simulink model "v1_0_3_sim_fsfc"  (R2024a)
settings: Solver=FixedStepAuto  StartTime=0.0  StopTime=inf  FixedStep=Ts_pwm  RelTol=1e-3
values from neighbouring files (symbols this model uses):
  A = [ -Rs/L,           0,                  0 ... (first row only)    [mcb_pmsm_fsfb_f28379d_param.m]    (also in v0_pmsm_fsfb_sim_for_flipsky_.m = [; v1_0_3_sim_param_fsfc.m = [)
  B = [ 1/L,  0 ... (first row only)    [mcb_pmsm_fsfb_f28379d_param.m]    (also in v0_pmsm_fsfb_sim_for_flipsky_.m = [; v1_0_3_sim_param_fsfc.m = [)
  Bv = pmsm.B    [mcb_pmsm_foc_qep_f28379d_SIUnit_data.m]    (also in mcb_pmsm_fsfb_f28379d_param.m = 2.636e-06; v0_pmsm_fsfb_sim_for_flipsky_.m = 9.444e-05; v1_0_3_sim_param_fsfc.m = 9.444e-05)
  C = [ 1, 0, 0 ... (first row only)    [mcb_pmsm_fsfb_f28379d_param.m]    (also in v0_pmsm_fsfb_sim_for_flipsky_.m = [; v1_0_3_sim_param_fsfc.m = [)
  J = 7.061e-6    (= 7.061e-06)    [mcb_pmsm_fsfb_f28379d_param.m]    (also in v0_pmsm_fsfb_sim_for_flipsky_.m = 0.00036179; v1_0_3_sim_param_fsfc.m = 0.00036179)
  Ki = -Ka_fsfb(2)    [mcb_pmsm_foc_qep_f28379d_SIUnit_data.m]    (also in mcb_pmsm_fsfb_f28379d_param.m = -K(:, n+1:end); v0_pmsm_fsfb_sim_for_flipsky_.m = -K(:, n+1:end); v1_0_3_sim_param_fsfc.m = -K(:, n+1:end))
  Kx = K(:, 1:n)    [mcb_pmsm_fsfb_f28379d_param.m]    (also in v0_pmsm_fsfb_sim_for_flipsky_.m; v1_0_3_sim_param_fsfc.m)
  L = Ld    (= 0.0002)    [mcb_pmsm_fsfb_f28379d_param.m]    (also in v0_pmsm_fsfb_sim_for_flipsky_.m = 0.0004; v1_0_3_sim_param_fsfc.m = 0.0013)
  Lambda_m = 0.01273    [mcb_pmsm_fsfb_f28379d_param.m]    (also in v0_pmsm_fsfb_sim_for_flipsky_.m = 0.0426; v1_0_3_sim_param_fsfc.m = 0.08627)
  P = 8    [mcb_pmsm_fsfb_f28379d_param.m]    (also in v0_pmsm_fsfb_sim_for_flipsky_.m; v1_0_3_sim_param_fsfc.m)
  Pk0 = 5e-4*diag([1e-3, 1e-2, 0.2, 0.01])    [v0_pmsm_fsfb_sim_for_flipsky_.m]    (also in v1_0_3_sim_param_fsfc.m)
  Qd = 1e-4*diag([0.5, 0.5, 5, 0.5])    [v0_pmsm_fsfb_sim_for_flipsky_.m]    (also in v1_0_3_sim_param_fsfc.m)
  R = Rs    (= 0.72)    [v0_pmsm_fsfb_sim_for_flipsky_.m]    (also in v1_0_3_sim_param_fsfc.m = 0.52)
  Rc = 56.33    [v0_pmsm_fsfb_sim_for_flipsky_.m]    (also in v1_0_3_sim_param_fsfc.m = 450)
  Rs = 0.3819    [mcb_pmsm_fsfb_f28379d_param.m]    (also in v0_pmsm_fsfb_sim_for_flipsky_.m = 0.72; v1_0_3_sim_param_fsfc.m = 0.52)
  Tc = 0.001    [v0_pmsm_fsfb_sim_for_flipsky_.m]    (also in v1_0_3_sim_param_fsfc.m)
  Ts = T_pwm    (= 5e-05)    [mcb_pmsm_foc_qep_f28379d_SIUnit_data.m]    (also in v0_pmsm_fsfb_sim_for_flipsky_.m = 0.0001; v1_0_3_sim_param_fsfc.m = 0.0001)
  Ts_ov = 1e-6    (= 1e-06)    [v0_pmsm_fsfb_sim_for_flipsky_.m]    (also in v1_0_3_sim_param_fsfc.m)
  Ts_pwm = 1/20000    (= 5e-05)    [mcb_pmsm_fsfb_f28379d_param.m]    (also in v0_pmsm_fsfb_sim_for_flipsky_.m = 0.0001; v1_0_3_sim_param_fsfc.m = 0.0001)
  Vdc = 24    [mcb_pmsm_fsfb_f28379d_param.m]    (also in v0_pmsm_fsfb_sim_for_flipsky_.m = 48*sqrt(3); v1_0_3_sim_param_fsfc.m = 150*sqrt(3))
  X03 = [0; 0; 0]    [v0_pmsm_fsfb_sim_for_flipsky_.m]    (also in v1_0_3_sim_param_fsfc.m)
  X04 = 1e-2*[1; 1; 1; 0]    [v0_pmsm_fsfb_sim_for_flipsky_.m]    (also in v1_0_3_sim_param_fsfc.m)
undefined symbols (not defined in the file or in its folder): Down, Up
libraries: spsMosfetLib x6, simulink x4, spsDCVoltageSourceLib x1, spsGroundLib x1, spsPermanentMagnetSynchronousMachineLib x1, spsThreePhaseVIMeasurementLib x1, spspowerguiLib x1, eeGeneralControl x1, spsSVPWMGenerator2LevelLib x1
(part 1 of 2)
settings Model: Creator=rotanakchhean  LastModifiedBy=rotanakchhean

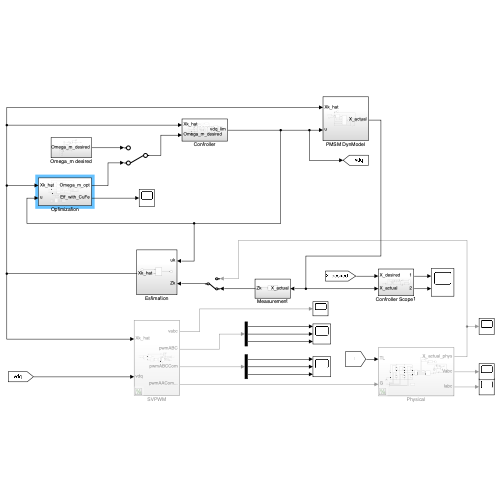
[thumbnail: Simulink's stored preview of the top-level diagram]
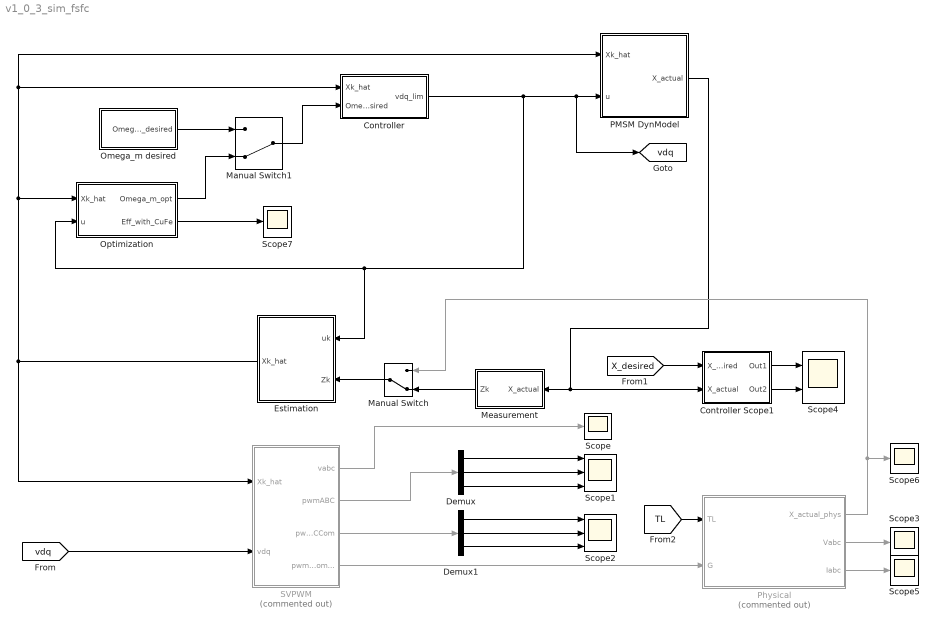
== system v1_0_3_sim_fsfc ==
  Controller : Subsystem
  Controller Scope1 : Subsystem
  Demux : Demux  Outputs=3
  Demux1 : Demux  Outputs=3
  Estimation : Subsystem
  Manual Switch : ManualSwitch  CurrentSetting=0
  Manual Switch1 : ManualSwitch  CurrentSetting=0
  Measurement : Subsystem
  Omega_m desired : Subsystem
  Optimization : Subsystem
  PMSM DynModel : Subsystem
  Physical : Subsystem  Commented=on
  SVPWM : Subsystem  Commented=on
  Scope{,3,5..7} (5 alike) : Scope
  Scope1 : Scope  NumInputPorts=3
  Scope2 : Scope  NumInputPorts=3
  Scope4 : Scope  NumInputPorts=2
  tag scope: vdq=global
  wires:
  Estimation/1(Xk_hat) -> Optimization/1(Xk_hat), PMSM DynModel/1(Xk_hat), Controller/1(Xk_hat), SVPWM/1(Xk_hat)
  SVPWM/1(vabc) -> Scope/1
  [vdq] -> SVPWM/2(vdq)
  Controller Scope1/2(Out2) -> Scope4/2
  Controller Scope1/1(Out1) -> Scope4/1
  [X_desired] -> Controller Scope1/1(X_desired)
  PMSM DynModel/1(X_actual) -> Measurement/1(X_actual), Controller Scope1/2(X_actual)
  SVPWM/2(pwmABC) -> Demux/1
  SVPWM/3(pwmABCCom) -> Demux1/1
  Demux/1 -> Scope1/1
  Demux/2 -> Scope1/2
  Demux/3 -> Scope1/3
  Demux1/1 -> Scope2/1
  Demux1/2 -> Scope2/2
  Demux1/3 -> Scope2/3
  SVPWM/4(pwmAACom...) -> Physical/2(G)
  [TL] -> Physical/1(TL)
  Physical/2(Vabc) -> Scope3/1
  Physical/3(Iabc) -> Scope5/1
  Physical/1(X_actual_phys) -> Manual Switch/1, Scope6/1
  Measurement/1(Zk) -> Manual Switch/2
  Manual Switch/1 -> Estimation/2(Zk)
  Optimization/2(Eff_with_CuFe) -> Scope7/1
  Controller/1(vdq_lim) -> Optimization/2(u), Estimation/1(uk), [vdq], PMSM DynModel/2(u)
  Omega_m desired/1(Omega_m_desired) -> Manual Switch1/1
  Optimization/1(Omega_m_opt) -> Manual Switch1/2
  Manual Switch1/1 -> Controller/2(Omega_m_desired)

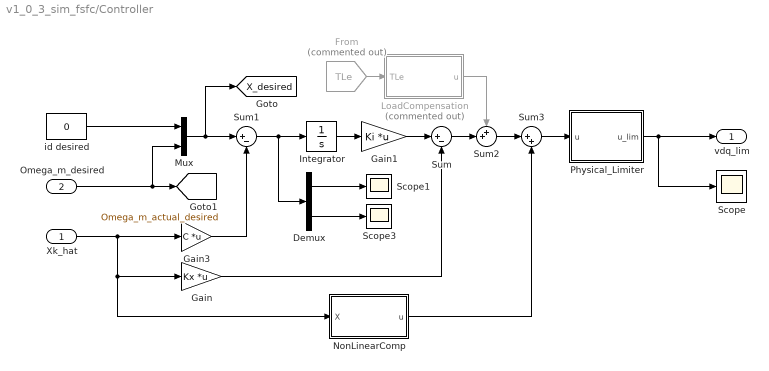
== system v1_0_3_sim_fsfc/Controller ==
  Xk_hat : Inport
  Omega_m_desired : Inport  Port=2
  Demux : Demux  Outputs=2
  From : From  Commented=on  GotoTag=TLe  TagVisibility=global
  Gain : Gain  Gain=Kx  Multiplication=Matrix(K*u)
  Gain1 : Gain  Gain=Ki  Multiplication=Matrix(K*u)
  Gain3 : Gain  Gain=C  Multiplication=Matrix(K*u)
  Integrator : Integrator
  LoadCompensation : MATLAB Function  Commented=on  TreatAsAtomicUnit=on
  Mux : Mux  Inputs=2
  NonLinearComp : MATLAB Function  TreatAsAtomicUnit=on
  Physical_Limiter : MATLAB Function  TreatAsAtomicUnit=on
  Scope : Scope
  Scope1 : Scope
  Scope3 : Scope
  Sum : Sum  Inputs=|+-
  Sum1 : Sum  Inputs=|+-
  Sum2 : Sum  Inputs=++|
  Sum3 : Sum  Inputs=|++
  id desired : Constant  Value=0
  vdq_lim : Outport
  tag scope: Omega_m_actual_desired=global, X_desired=global
  wires:
  Gain1/1 -> Sum/1
  NonLinearComp/1(u) -> Sum3/2
  Gain/1 -> Sum/2
  Sum1/1 -> Integrator/1, Demux/1
  Sum/1 -> Sum2/2
  Integrator/1 -> Gain1/1
  Gain3/1 -> Sum1/2
  Omega_m_desired/1 -> Mux/2, [Omega_m_actual_desired]
  id desired/1 -> Mux/1
  Physical_Limiter/1(u_lim) -> Scope/1, vdq_lim/1
  Sum3/1 -> Physical_Limiter/1(u)
  LoadCompensation/1(u) -> Sum2/1
  Xk_hat/1 -> Gain/1, NonLinearComp/1(X), Gain3/1
  Sum2/1 -> Sum3/1
  Demux/1 -> Scope1/1
  From/1 -> LoadCompensation/1(TLe)
  Demux/2 -> Scope3/1
  Mux/1 -> [X_desired], Sum1/1

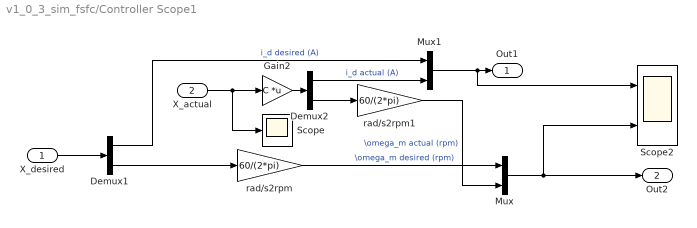
== system v1_0_3_sim_fsfc/Controller Scope1 ==
  X_desired : Inport
  X_actual : Inport  Port=2
  Demux1 : Demux  Outputs=2
  Demux2 : Demux  Outputs=2
  Gain2 : Gain  Gain=C  Multiplication=Matrix(K*u)
  Mux : Mux  Inputs=2
  Mux1 : Mux  Inputs=2
  Scope : Scope
  Scope2 : Scope  NumInputPorts=2
  rad/s2rpm : Gain  Gain=60/(2*pi)
  rad/s2rpm1 : Gain  Gain=60/(2*pi)
  Out1 : Outport
  Out2 : Outport  Port=2
  wires:
  X_actual/1 -> Scope/1, Gain2/1
  Demux1/1 -> Mux1/1  "i_d desired (A)"
  Demux2/1 -> Mux1/2  "i_d actual (A)"
  Gain2/1 -> Demux2/1
  Mux1/1 -> Scope2/1, Out1/1
  X_desired/1 -> Demux1/1
  Demux2/2 -> rad/s2rpm1/1
  Demux1/2 -> rad/s2rpm/1
  Mux/1 -> Scope2/2, Out2/1
  rad/s2rpm/1 -> Mux/1  "\\omega_m desired (rpm)"
  rad/s2rpm1/1 -> Mux/2  "\\omega_m actual (rpm)"

== system v1_0_3_sim_fsfc/Estimation ==
  uk : Inport
  Zk : Inport  Port=2
  EKF Estimation : Subsystem
  Xk_hat : Outport
  wires:
  EKF Estimation/1(Xk_hat) -> Xk_hat/1
  Zk/1 -> EKF Estimation/2(Zk)
  uk/1 -> EKF Estimation/1(uk)

== system v1_0_3_sim_fsfc/Measurement ==
  X_actual : Inport
  Measurement Noise : Subsystem
  Zk : Outport
  wires:
  X_actual/1 -> Measurement Noise/1(In2)
  Measurement Noise/1(Zk) -> Zk/1

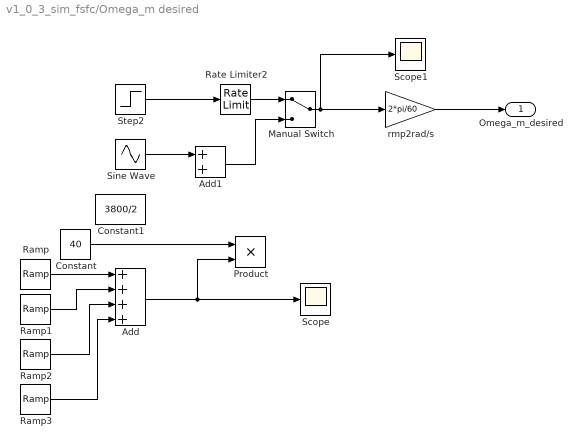
== system v1_0_3_sim_fsfc/Omega_m desired ==
  Add : Sum  Inputs=++++
  Add1 : Sum
  Constant : Constant  Value=40
  Constant1 : Constant  Value=3800/2
  Manual Switch : ManualSwitch
  Product : Product
  Ramp : simulink/Sources/Ramp  slope=1  start=5  InitialOutput=0
  Ramp1 : simulink/Sources/Ramp  slope=-1  start=15  InitialOutput=0
  Ramp2 : simulink/Sources/Ramp  slope=-1  start=35  InitialOutput=0
  Ramp3 : simulink/Sources/Ramp  slope=1  start=45  InitialOutput=0
  Rate Limiter2 : RateLimiter  RisingSlewLimit=700  FallingSlewLimit=-700  SampleTimeMode=inherited
  Scope : Scope
  Scope1 : Scope
  Sine Wave : Sin  Amplitude=3800  Frequency=2*pi*0.25  SampleTime=0
  Step2 : Step  Time=0  After=2200  SampleTime=0
  rmp2rad/s : Gain  Gain=2*pi/60
  Omega_m_desired : Outport
  wires:
  Rate Limiter2/1 -> Manual Switch/1
  rmp2rad/s/1 -> Omega_m_desired/1
  Sine Wave/1 -> Add1/1
  Step2/1 -> Rate Limiter2/1
  Ramp/1 -> Add/1
  Ramp1/1 -> Add/2
  Ramp2/1 -> Add/3
  Add/1 -> Product/2, Scope/1
  Ramp3/1 -> Add/4
  Constant/1 -> Product/1
  Manual Switch/1 -> Scope1/1, rmp2rad/s/1
  Add1/1 -> Manual Switch/2

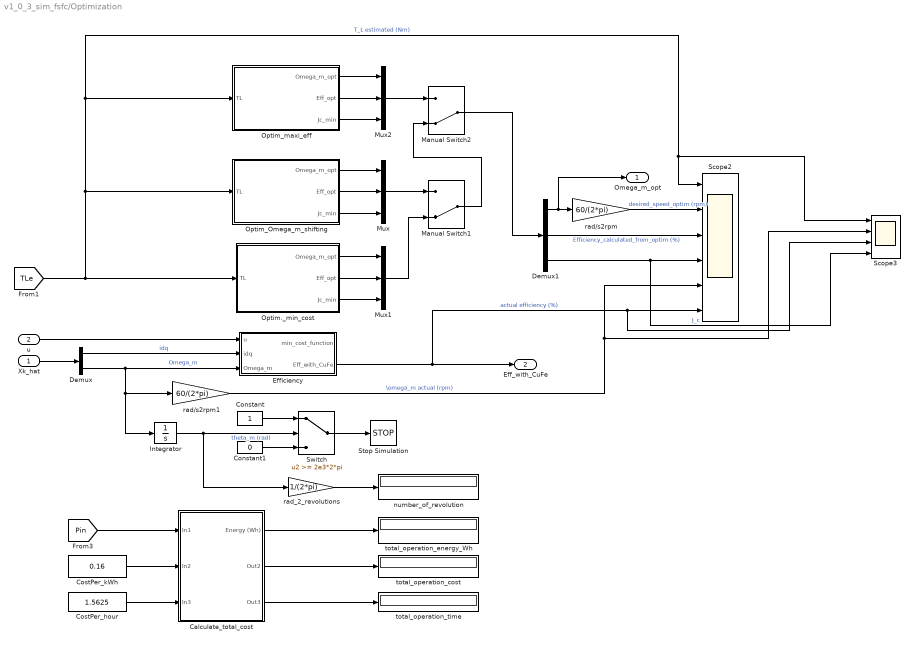
== system v1_0_3_sim_fsfc/Optimization ==
  Xk_hat : Inport
  u : Inport  Port=2
  Calculate_total_cost : Subsystem
  Constant : Constant
  Constant1 : Constant  Value=0
  CostPer_hour : Constant  Value=1.5625
  CostPer_kWh : Constant  Value=0.16
  Demux : Demux  Outputs=[2, 1]
  Demux1 : Demux  Outputs=3
  Efficiency : Subsystem
  Integrator : Integrator
  Manual Switch1 : ManualSwitch  CurrentSetting=0
  Manual Switch2 : ManualSwitch  CurrentSetting=0
  Mux : Mux  Inputs=3
  Mux1 : Mux  Inputs=3
  Mux2 : Mux  Inputs=3
  Optim._min_cost : MATLAB Function  TreatAsAtomicUnit=on
  Optim_Omega_m_shifting : MATLAB Function  TreatAsAtomicUnit=on
  Optim_maxi_eff : MATLAB Function  TreatAsAtomicUnit=on
  Scope2 : Scope  NumInputPorts=6
  Scope3 : Scope  NumInputPorts=4
  Stop Simulation : Stop
  Switch : Switch  Threshold=2e3*2*pi  SaturateOnIntegerOverflow=off  InputSameDT=off
  number_of_revolution : Display
  rad/s2rpm : Gain  Gain=60/(2*pi)
  rad/s2rpm1 : Gain  Gain=60/(2*pi)
  rad_2_revolutions : Gain  Gain=1/(2*pi)
  total_operation_cost : Display
  total_operation_energy_Wh : Display
  total_operation_time : Display
  Omega_m_opt : Outport
  Eff_with_CuFe : Outport  Port=2
  wires:
  Xk_hat/1 -> Demux/1
  u/1 -> Efficiency/1(u)
  Demux/1 -> Efficiency/2(idq)  "idq"
  Demux/2 -> Efficiency/3(Omega_m), Integrator/1, rad/s2rpm1/1  "Omega_m"
  rad/s2rpm/1 -> Scope2/2  "desired_speed_optim (rpm)"
  Efficiency/2(Eff_with_CuFe) -> Scope3/3, Scope2/6, Eff_with_CuFe/1  "actual efficiency (%)"
  Demux1/1 -> rad/s2rpm/1, Omega_m_opt/1
  [TLe] -> Optim._min_cost/1(TL), Optim_Omega_m_shifting/1(TL), Scope2/1, Scope3/1, Optim_maxi_eff/1(TL)  "T_L estimated (Nm)"
  rad/s2rpm1/1 -> Scope2/5, Scope3/2  "\\omega_m actual (rpm)"
  Integrator/1 -> Switch/2, rad_2_revolutions/1  "theta_m (rad)"
  Constant1/1 -> Switch/3
  Constant/1 -> Switch/1
  Calculate_total_cost/2(Out2) -> total_operation_cost/1
  [Pin] -> Calculate_total_cost/1(In1)
  CostPer_kWh/1 -> Calculate_total_cost/2(In2)
  CostPer_hour/1 -> Calculate_total_cost/3(In3)
  Calculate_total_cost/1(Energy (Wh)) -> total_operation_energy_Wh/1
  Calculate_total_cost/3(Out3) -> total_operation_time/1
  Optim_Omega_m_shifting/3(Jc_min) -> Mux/3
  Optim_Omega_m_shifting/2(Eff_opt) -> Mux/2
  Optim._min_cost/2(Eff_opt) -> Mux1/2
  Optim._min_cost/1(Omega_m_opt) -> Mux1/1
  Optim._min_cost/3(Jc_min) -> Mux1/3
  Mux/1 -> Manual Switch1/1
  Mux1/1 -> Manual Switch1/2
  Optim_Omega_m_shifting/1(Omega_m_opt) -> Mux/1
  Demux1/3 -> Scope3/4, Scope2/4  "J_c"
  rad_2_revolutions/1 -> number_of_revolution/1
  Optim_maxi_eff/1(Omega_m_opt) -> Mux2/1
  Optim_maxi_eff/2(Eff_opt) -> Mux2/2
  Optim_maxi_eff/3(Jc_min) -> Mux2/3
  Mux2/1 -> Manual Switch2/1
  Manual Switch1/1 -> Manual Switch2/2
  Manual Switch2/1 -> Demux1/1
  Demux1/2 -> Scope2/3  "Efficiency_calculated_from_optim (%)"
  Switch/1 -> Stop Simulation/1

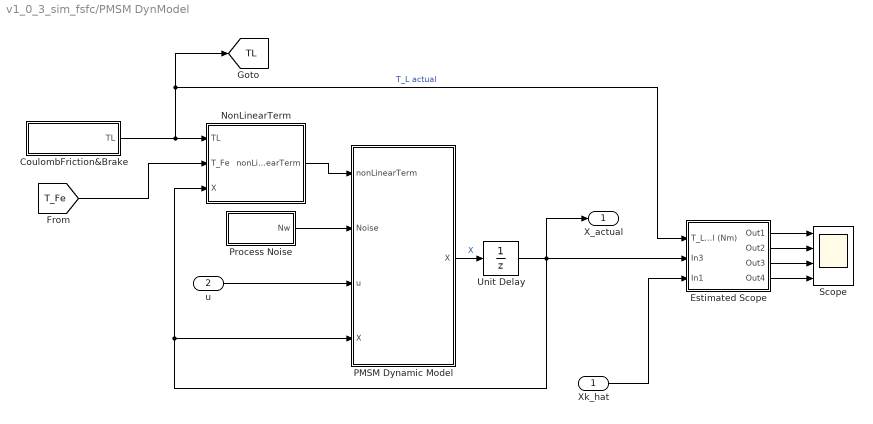
== system v1_0_3_sim_fsfc/PMSM DynModel ==
  Xk_hat : Inport
  u : Inport  Port=2
  CoulombFriction&Brake : Subsystem
  Estimated Scope : Subsystem
  NonLinearTerm : MATLAB Function  TreatAsAtomicUnit=on
  PMSM Dynamic Model : MATLAB Function  TreatAsAtomicUnit=on
  Process Noise : Subsystem
  Scope : Scope  NumInputPorts=4
  Unit Delay : UnitDelay  InitialCondition=X03  SampleTime=-1  HasFrameUpgradeWarning=on
  X_actual : Outport
  tag scope: TL=global
  wires:
  Xk_hat/1 -> Estimated Scope/3(In1)
  Estimated Scope/4(Out4) -> Scope/4
  Estimated Scope/2(Out2) -> Scope/2
  Estimated Scope/1(Out1) -> Scope/1
  Unit Delay/1 -> NonLinearTerm/3(X), PMSM Dynamic Model/4("X "), X_actual/1, Estimated Scope/2(In3)
  Process Noise/1(Nw) -> PMSM Dynamic Model/2(Noise)
  PMSM Dynamic Model/1(X) -> Unit Delay/1  "X"
  NonLinearTerm/1(nonLinearTerm) -> PMSM Dynamic Model/1(nonLinearTerm)
  Estimated Scope/3(Out3) -> Scope/3
  CoulombFriction&Brake/1(TL) -> [TL], Estimated Scope/1(T_L actual (Nm)), NonLinearTerm/1(TL)  "T_L actual"
  u/1 -> PMSM Dynamic Model/3(u)
  [T_Fe] -> NonLinearTerm/2(T_Fe)

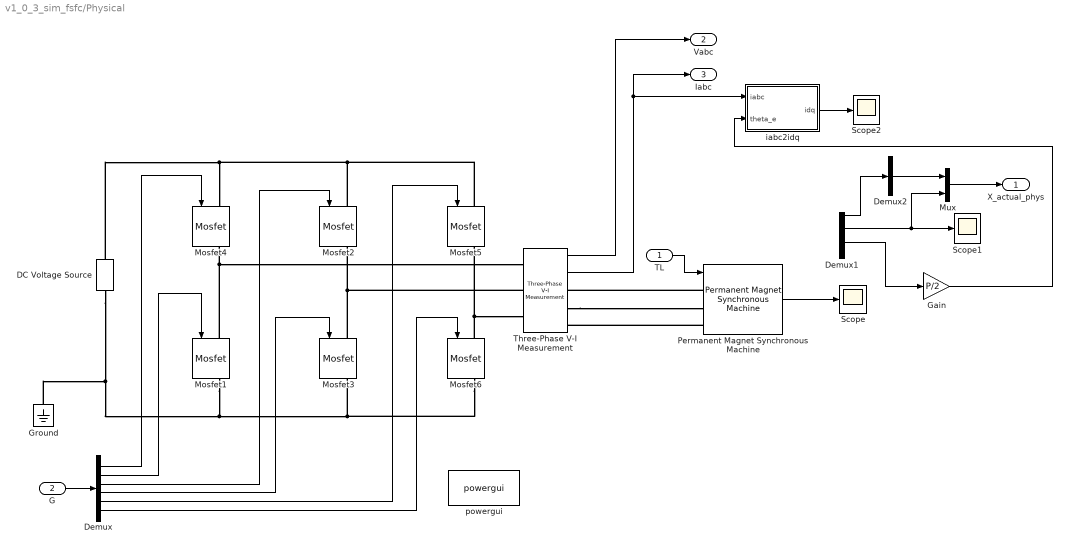
== system v1_0_3_sim_fsfc/Physical ==
  TL : Inport
  G : Inport  Port=2
  DC Voltage Source : spsDCVoltageSourceLib/DC Voltage Source  Amplitude=Vdc  Measurements=None
  Demux : Demux  Outputs=6
  Demux1 : Demux  Outputs=[10, 1, 1, 1]
  Demux2 : Demux  Outputs=[3, 2, 5]
  Gain : Gain  Gain=P/2
  Ground : spsGroundLib/Ground  LConnTagsString=a
  Mosfet{1..6} (6 alike) : spsMosfetLib/Mosfet  Ron=0.001  Lon=0  Rd=0.001  Vfd=0.6  IC=0  Rs=1e5  Cs=inf  Measurements=on
  Mux : Mux  Inputs=2
  Permanent Magnet Synchronous Machine : spsPermanentMagnetSynchronousMachineLib/Permanent Magnet Synchronous Machine  NbPhases=3  FluxDistribution=Sinusoidal  RotorType=Round  MechanicalLoad=Torque Tm  PresetModel=No  ShowDetailedParameters=on  MeasurementBus=off  Resistance=R  Inductance=8.5e-3  dqInductances=[8.5e-3,8.5e-3]  La=L  MachineConstant=Flux linkage established by magnets (V.s)  Flux=Lambda_m  VoltageCst=62.5906  TorqueCst=0.51762  Flat=120  Mechanical=[J Bv P/2 1e-3]  PolePairs=4  InitialConditions=[0,0, 0,0]  InitialConditions5ph=[0 0 0 0 0 0]  RefAngle=90 degrees behind phase A axis (modified Park)  IterativeDiscreteModel=Trapezoidal non iterative  TsBlock=-1  TsPowergui=0
  Scope : Scope
  Scope1 : Scope
  Scope2 : Scope
  Three-Phase V-I Measurement : spsThreePhaseVIMeasurementLib/Three-Phase V-I Measurement  VoltageMeasurement=phase-to-phase  SetLabelV=off  LabelV=Vabc  Vpu=off  VpuLL=off  CurrentMeasurement=yes  SetLabelI=off  LabelI=Iabc  Ipu=off  Pbase=100e6  Vbase=500e3  OutputType=Complex  PhasorSimulation=off  PSBequivalent=0
  iabc2idq : Subsystem
  powergui : spspowerguiLib/powergui  Priority=1  SimulationMode=Continuous  SampleTime=50e-6  frequency=60  Iterations=50  frequencyindice=0  Pbase=100e6  ErrMax=1e-4  UnitsV=kV  UnitsW=MW  buscounter=0  FunctionMessages=off  echomessages=off  EnableUseOfTLC=off  CurrentSourceSwitches=off  DisableSnubberDevices=off  DisableRonSwitches=off  DisableVfSwitches=off  DisplayEquations=off  AutomaticDiscreteSolvers=off  SolverType=Tustin/Backward Euler (TBE)  Interpol=off  ExternalGateDelay=off  methode=off  Ts=100  x0status=blocks  SPID=on  SwTol=0  HookPort=off  NonlinearTolerance=1e-4  nMaxIteration=100  ContinueOnMaxIteration=off  RestoreLinks=warning  ResistiveCurrentMeasurement=off  Frange=[0:2:500]  Ylog=off  Xlog=on  ShowGrid=off  save=off  variable=ZData  structure=0  ZoomFFT=off  StartTime=0.0  cycles=1  DisplayStyle=1  fundamental=60  FreqAxis=off  MaxFrequency=1000  frequencyindicesteady=1  RmsSteady=1  display=off
  X_actual_phys : Outport
  Vabc : Outport  Port=2
  Iabc : Outport  Port=3
  wires:
  G/1 -> Demux/1
  Demux/1 -> Mosfet4/1
  Demux/2 -> Mosfet1/1
  Demux/3 -> Mosfet2/1
  Demux/4 -> Mosfet3/1
  Demux/5 -> Mosfet5/1
  Demux/6 -> Mosfet6/1
  TL/1 -> Permanent Magnet Synchronous Machine/1
  Three-Phase V-I Measurement/2 -> Iabc/1, iabc2idq/1(iabc)
  Three-Phase V-I Measurement/1 -> Vabc/1
  Permanent Magnet Synchronous Machine/1 -> Scope/1
  Demux1/2 -> Scope1/1, Mux/2
  Demux1/3 -> Gain/1
  Gain/1 -> iabc2idq/2(theta_e)
  iabc2idq/1(idq) -> Scope2/1
  Demux1/1 -> Demux2/1
  Demux2/2 -> Mux/1
  Mux/1 -> X_actual_phys/1
  connections:
  DC Voltage Source/RConn1 -- Mosfet5/LConn1 -- Mosfet2/LConn1 -- Mosfet4/LConn1
  Mosfet1/RConn1 -- Ground/LConn1 -- DC Voltage Source/LConn1 -- Mosfet3/RConn1 -- Mosfet6/RConn1
  Mosfet3/LConn1 -- Three-Phase V-I Measurement/LConn2 -- Mosfet2/RConn1
  Mosfet6/LConn1 -- Mosfet5/RConn1 -- Three-Phase V-I Measurement/LConn3
  Mosfet1/LConn1 -- Mosfet4/RConn1 -- Three-Phase V-I Measurement/LConn1
  Permanent Magnet Synchronous Machine/LConn1 -- Three-Phase V-I Measurement/RConn1
  Three-Phase V-I Measurement/RConn2 -- Permanent Magnet Synchronous Machine/LConn2
  Permanent Magnet Synchronous Machine/LConn3 -- Three-Phase V-I Measurement/RConn3

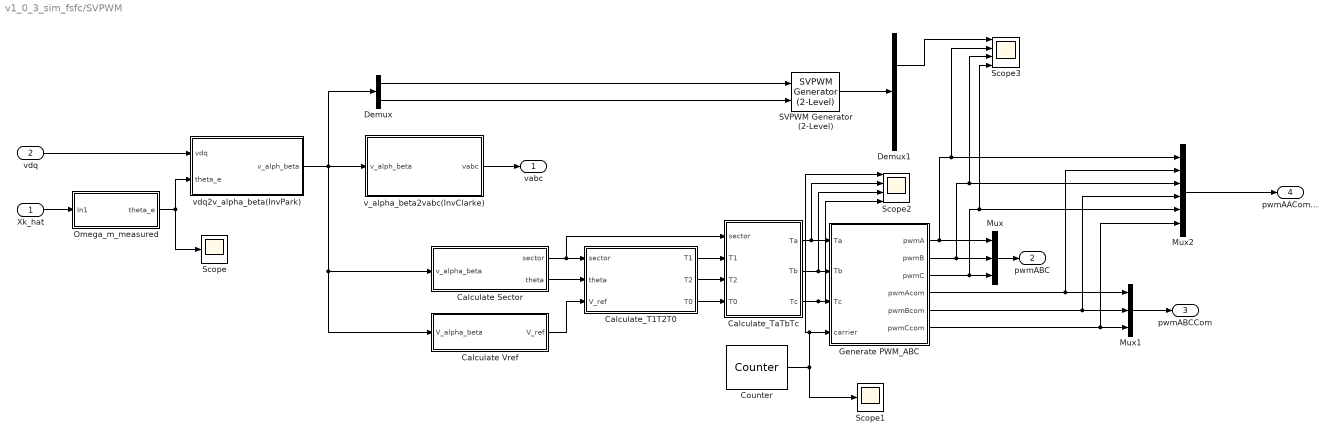
== system v1_0_3_sim_fsfc/SVPWM ==
  Xk_hat : Inport
  vdq : Inport  Port=2
  Calculate Sector : MATLAB Function  TreatAsAtomicUnit=on
  "Calculate Vref " : MATLAB Function  TreatAsAtomicUnit=on
  Calculate_T1T2T0 : MATLAB Function  TreatAsAtomicUnit=on
  Calculate_TaTbTc : MATLAB Function  TreatAsAtomicUnit=on
  Counter : eeGeneralControl/Counter  CarrCount=Up-Down  Range=[0 1]  Tper=Ts_pwm/2  Tdelay=0  Ts=Ts_ov
      settings: LibrarySourceBlock=ee_sl_lib/General Control/Counter
  Demux : Demux  Outputs=2
  Demux1 : Demux  Outputs=6
  Generate PWM_ABC : MATLAB Function  TreatAsAtomicUnit=on
  Mux : Mux  Inputs=3
  Mux1 : Mux  Inputs=3
  Mux2 : Mux  Inputs=6
  Omega_m_measured : Subsystem
  SVPWM Generator (2-Level) : spsSVPWMGenerator2LevelLib/SVPWM Generator (2-Level)  InputType=alpha-beta components  SwitchingPattern=Pattern #1  Fc=1e4  ParUref=[0.8 -30 50]  Ts=0
  Scope : Scope
  Scope1 : Scope
  Scope2 : Scope  NumInputPorts=4
  Scope3 : Scope  NumInputPorts=4
  v_alpha_beta2vabc(InvClarke) : MATLAB Function  TreatAsAtomicUnit=on
  vdq2v_alpha_beta(InvPark) : MATLAB Function  TreatAsAtomicUnit=on
  vabc : Outport
  pwmABC : Outport  Port=2
  pwmABCCom : Outport  Port=3
  pwmAACom... : Outport  Port=4
  wires:
  vdq/1 -> vdq2v_alpha_beta(InvPark)/1(vdq)
  Omega_m_measured/1(theta_e) -> Scope/1, vdq2v_alpha_beta(InvPark)/2(theta_e)
  v_alpha_beta2vabc(InvClarke)/1(vabc) -> vabc/1
  Xk_hat/1 -> Omega_m_measured/1(In1)
  Calculate_T1T2T0/1(T1) -> Calculate_TaTbTc/2(T1)
  "Calculate Vref "/1(V_ref) -> Calculate_T1T2T0/3(V_ref)
  Calculate_T1T2T0/2(T2) -> Calculate_TaTbTc/3(T2)
  Calculate_T1T2T0/3(T0) -> Calculate_TaTbTc/4(T0)
  Calculate_TaTbTc/1(Ta) -> Scope2/2, Generate PWM_ABC/1(Ta)
  Calculate_TaTbTc/2(Tb) -> Scope2/3, Generate PWM_ABC/2(Tb)
  Calculate_TaTbTc/3(Tc) -> Scope2/4, Generate PWM_ABC/3(Tc)
  Counter/1 -> Scope1/1, Generate PWM_ABC/4(carrier), Scope2/1
  Calculate Sector/2(theta) -> Calculate_T1T2T0/2(theta)
  Calculate Sector/1(sector) -> Calculate_T1T2T0/1(sector), Calculate_TaTbTc/1(sector)
  Generate PWM_ABC/1(pwmA) -> Mux/1, Mux2/1, Scope3/2
  Generate PWM_ABC/2(pwmB) -> Mux/2, Mux2/3, Scope3/3
  Generate PWM_ABC/3(pwmC) -> Mux/3, Scope3/4, Mux2/5
  Generate PWM_ABC/5(pwmBcom) -> Mux1/2, Mux2/4
  Generate PWM_ABC/6(pwmCcom) -> Mux1/3, Mux2/6
  Generate PWM_ABC/4(pwmAcom) -> Mux1/1, Mux2/2
  Mux1/1 -> pwmABCCom/1
  Mux/1 -> pwmABC/1
  Demux/1 -> SVPWM Generator (2-Level)/1
  Demux/2 -> SVPWM Generator (2-Level)/2
  vdq2v_alpha_beta(InvPark)/1(v_alph_beta) -> "Calculate Vref "/1(V_alpha_beta), Calculate Sector/1(v_alpha_beta), v_alpha_beta2vabc(InvClarke)/1(v_alph_beta), Demux/1
  SVPWM Generator (2-Level)/1 -> Demux1/1
  Demux1/2 -> Scope3/1
  Mux2/1 -> pwmAACom.../1

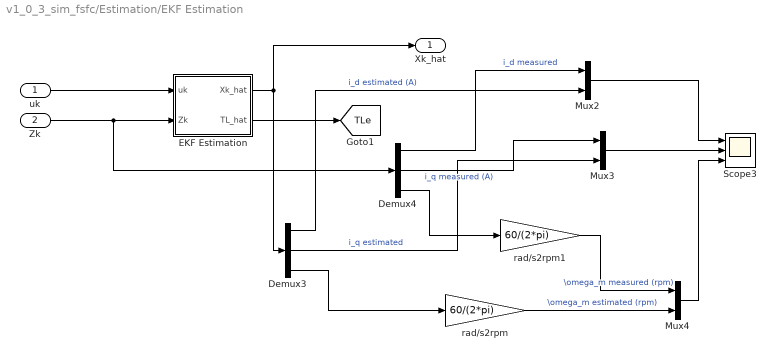
== system v1_0_3_sim_fsfc/Estimation/EKF Estimation ==
  uk : Inport
  Zk : Inport  Port=2
  Demux3 : Demux  Outputs=3
  Demux4 : Demux  Outputs=3
  EKF Estimation : Subsystem
  Mux2 : Mux  Inputs=2
  Mux3 : Mux  Inputs=2
  Mux4 : Mux  Inputs=2
  Scope3 : Scope  NumInputPorts=3
  rad/s2rpm : Gain  Gain=60/(2*pi)
  rad/s2rpm1 : Gain  Gain=60/(2*pi)
  Xk_hat : Outport
  tag scope: TLe=global
  wires:
  uk/1 -> EKF Estimation/1(uk)
  Demux3/3 -> rad/s2rpm/1
  EKF Estimation/1(Xk_hat) -> Xk_hat/1, Demux3/1
  Demux4/2 -> Mux3/1  "i_q measured (A)"
  Mux3/1 -> Scope3/2
  Demux3/1 -> Mux2/2  "i_d estimated (A)"
  Zk/1 -> Demux4/1, EKF Estimation/2(Zk)
  Demux4/3 -> rad/s2rpm1/1
  Mux2/1 -> Scope3/1
  Demux3/2 -> Mux3/2  "i_q estimated"
  EKF Estimation/2(TL_hat) -> [TLe]
  Demux4/1 -> Mux2/1  "i_d measured"
  Mux4/1 -> Scope3/3
  rad/s2rpm/1 -> Mux4/2  "\\omega_m estimated (rpm)"
  rad/s2rpm1/1 -> Mux4/1  "\\omega_m measured (rpm)"

== system v1_0_3_sim_fsfc/Measurement/Measurement Noise ==
  In2 : Inport
  Constant1 : Constant  Value=0.5
  Constant2 : Constant  Value=0.5
  Constant3 : Constant  Value=2
  "Measurement Noise " : MATLAB Function  TreatAsAtomicUnit=on
  Sum4 : Sum  Inputs=|++
  Zk : Outport
  wires:
  "Measurement Noise "/1(Nv) -> Sum4/2
  Constant2/1 -> "Measurement Noise "/2(Viq)
  Constant1/1 -> "Measurement Noise "/1(Vid)
  Constant3/1 -> "Measurement Noise "/3(Vwm)
  Sum4/1 -> Zk/1
  In2/1 -> Sum4/1

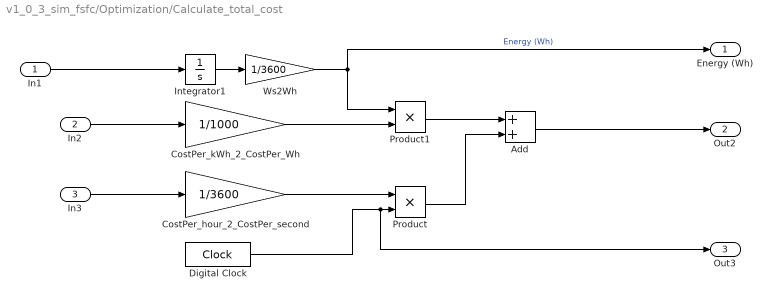
== system v1_0_3_sim_fsfc/Optimization/Calculate_total_cost ==
  In1 : Inport
  In2 : Inport  Port=2
  In3 : Inport  Port=3
  Add : Sum
  CostPer_hour_2_CostPer_second : Gain  Gain=1/3600
  CostPer_kWh_2_CostPer_Wh : Gain  Gain=1/1000
  Digital Clock : DigitalClock
  Integrator1 : Integrator
  Product : Product
  Product1 : Product
  Ws2Wh : Gain  Gain=1/3600
  Energy (Wh) : Outport
  Out2 : Outport  Port=2
  Out3 : Outport  Port=3
  wires:
  In1/1 -> Integrator1/1
  Add/1 -> Out2/1
  In3/1 -> CostPer_hour_2_CostPer_second/1
  CostPer_kWh_2_CostPer_Wh/1 -> Product1/2
  In2/1 -> CostPer_kWh_2_CostPer_Wh/1
  CostPer_hour_2_CostPer_second/1 -> Product/1
  Integrator1/1 -> Ws2Wh/1
  Product/1 -> Add/2
  Product1/1 -> Add/1
  Ws2Wh/1 -> Energy (Wh)/1, Product1/1  "Energy (Wh)"
  Digital Clock/1 -> Out3/1, Product/2

== system v1_0_3_sim_fsfc/Optimization/Efficiency ==
  u : Inport
  idq : Inport  Port=2
  Omega_m : Inport  Port=3
  Divide : Product  Inputs=*/
  MATLAB Function : MATLAB Function  TreatAsAtomicUnit=on
  Pin : Subsystem
  Pout : Subsystem
  Pout_hassan : Subsystem  Commented=on
  Scope : Scope
  min_cost_function : Outport
  Eff_with_CuFe : Outport  Port=2
  tag scope: Pin=global
  wires:
  idq/1 -> Pout/2(idq), Pin/1(idq)
  u/1 -> Pin/2(u)
  Pin/1(Pin) -> [Pin], Divide/2, Pout/3(Pin)
  Pout/1(Pout) -> Divide/1
  Divide/1 -> MATLAB Function/1("Eff ")
  Omega_m/1 -> Pout/1(Omega_m)
  MATLAB Function/1(Eff) -> Scope/1, Eff_with_CuFe/1

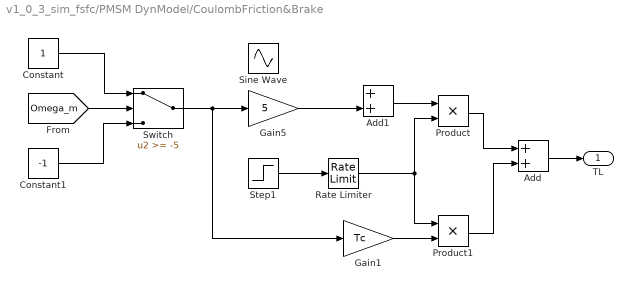
== system v1_0_3_sim_fsfc/PMSM DynModel/CoulombFriction&Brake ==
  Add : Sum
  Add1 : Sum
  Constant : Constant
  Constant1 : Constant  Value=-1
  Gain1 : Gain  Gain=Tc
  Gain5 : Gain  Gain=5
  Product : Product
  Product1 : Product
  Rate Limiter : RateLimiter  RisingSlewLimit=0.2  FallingSlewLimit=-0.2  SampleTimeMode=inherited
  Sine Wave : Sin  Amplitude=2  Frequency=2*pi*0.1  SampleTime=0
  Step1 : Step  Before=1  SampleTime=0
  Switch : Switch  Threshold=-5  SaturateOnIntegerOverflow=off  InputSameDT=off
  TL : Outport
  wires:
  Product/1 -> Add/1
  Switch/1 -> Gain5/1, Gain1/1
  Step1/1 -> Rate Limiter/1
  Gain1/1 -> Product1/2
  Product1/1 -> Add/2
  Add/1 -> TL/1
  Add1/1 -> Product/1
  Constant/1 -> Switch/1
  Constant1/1 -> Switch/3
  [Omega_m] -> Switch/2
  Rate Limiter/1 -> Product/2, Product1/1
  Gain5/1 -> Add1/2

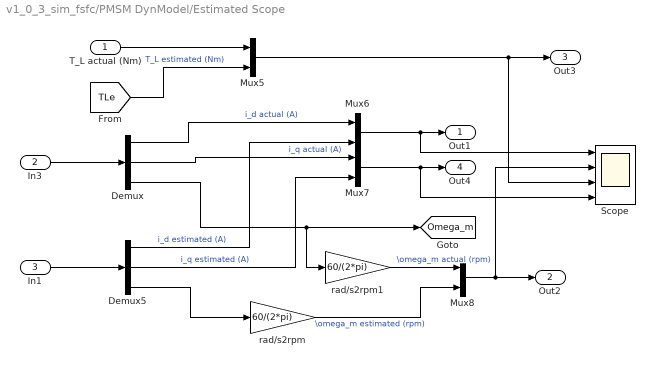
== system v1_0_3_sim_fsfc/PMSM DynModel/Estimated Scope ==
  T_L actual (Nm) : Inport
  In3 : Inport  Port=2
  In1 : Inport  Port=3
  Demux : Demux  Outputs=3
  Demux5 : Demux  Outputs=3
  Mux{5..8} (4 alike) : Mux  Inputs=2
  Scope : Scope  NumInputPorts=4
  rad/s2rpm : Gain  Gain=60/(2*pi)
  rad/s2rpm1 : Gain  Gain=60/(2*pi)
  Out1 : Outport
  Out2 : Outport  Port=2
  Out3 : Outport  Port=3
  Out4 : Outport  Port=4
  tag scope: Omega_m=global
  wires:
  In1/1 -> Demux5/1
  Demux5/3 -> rad/s2rpm/1
  [TLe] -> Mux5/2  "T_L estimated (Nm)"
  Mux6/1 -> Scope/1, Out1/1
  Mux5/1 -> Scope/3, Out3/1
  In3/1 -> Demux/1
  Demux/3 -> [Omega_m], rad/s2rpm1/1
  T_L actual (Nm)/1 -> Mux5/1
  Demux5/2 -> Mux7/2  "i_q estimated (A)"
  Demux5/1 -> Mux6/2  "i_d estimated (A)"
  Mux7/1 -> Scope/4, Out4/1
  Mux8/1 -> Scope/2, Out2/1
  Demux/1 -> Mux6/1  "i_d actual (A)"
  Demux/2 -> Mux7/1  "i_q actual (A)"
  rad/s2rpm/1 -> Mux8/2  "\\omega_m estimated (rpm)"
  rad/s2rpm1/1 -> Mux8/1  "\\omega_m actual (rpm)"

== system v1_0_3_sim_fsfc/PMSM DynModel/Process Noise ==
  Constant4 : Constant  Value=0.2e-4
  Constant5 : Constant  Value=0.2e-4
  Constant6 : Constant  Value=2e-4
  Process Noise : MATLAB Function  TreatAsAtomicUnit=on
  Nw : Outport
  wires:
  Constant5/1 -> Process Noise/2(Viq)
  Process Noise/1(Nw) -> Nw/1
  Constant4/1 -> Process Noise/1(Vid)
  Constant6/1 -> Process Noise/3(Vwm)

== system v1_0_3_sim_fsfc/Physical/iabc2idq ==
  iabc : Inport
  theta_e : Inport  Port=2
  i_alpha_beta2idq(FPark) : MATLAB Function  TreatAsAtomicUnit=on
  iabc2i_alpha_beta(FClarke) : MATLAB Function  TreatAsAtomicUnit=on
  idq : Outport
  wires:
  iabc/1 -> iabc2i_alpha_beta(FClarke)/1(iabc)
  iabc2i_alpha_beta(FClarke)/1(i_alpha_beta) -> i_alpha_beta2idq(FPark)/1(i_alpha_beta)
  i_alpha_beta2idq(FPark)/1(idq) -> idq/1
  theta_e/1 -> i_alpha_beta2idq(FPark)/2(theta_e)

== system v1_0_3_sim_fsfc/SVPWM/Omega_m_measured ==
  In1 : Inport
  Integrator : Integrator
  idqwm2wm : Gain  Gain=[0 0 1]  Multiplication=Matrix(K*u)
  wm2we : Gain  Gain=P/2
  theta_e : Outport
  wires:
  In1/1 -> idqwm2wm/1
  idqwm2wm/1 -> wm2we/1
  wm2we/1 -> Integrator/1
  Integrator/1 -> theta_e/1

== system v1_0_3_sim_fsfc/Estimation/EKF Estimation/EKF Estimation ==
  uk : Inport
  Zk : Inport  Port=2
  Demux : Demux
  MeasurementUpdateCorrect : MATLAB Function  TreatAsAtomicUnit=on
  Mux : Mux  Inputs=3
  TimeUpdatePredict : MATLAB Function  TreatAsAtomicUnit=on
  Unit Delay : UnitDelay  InitialCondition=Pk0  SampleTime=-1  HasFrameUpgradeWarning=on
  Unit Delay1 : UnitDelay  InitialCondition=X04  SampleTime=-1  HasFrameUpgradeWarning=on
  Unit Delay2 : UnitDelay  SampleTime=-1  HasFrameUpgradeWarning=on
  Xk_hat : Outport
  TL_hat : Outport  Port=2
  wires:
  uk/1 -> Unit Delay2/1
  TimeUpdatePredict/1(Pk1_p) -> MeasurementUpdateCorrect/2(Pk1_p)
  TimeUpdatePredict/2(Xk1_p) -> MeasurementUpdateCorrect/3(Xk1_p)
  Zk/1 -> MeasurementUpdateCorrect/1(Zk)
  MeasurementUpdateCorrect/2(Pk) -> Unit Delay/1
  Unit Delay/1 -> TimeUpdatePredict/3(Pk)
  MeasurementUpdateCorrect/1(Xk) -> Unit Delay1/1
  Unit Delay1/1 -> Demux/1, TimeUpdatePredict/2(Xk)
  Demux/3 -> Mux/3
  Demux/2 -> Mux/2
  Demux/1 -> Mux/1
  Mux/1 -> Xk_hat/1
  Demux/4 -> TL_hat/1
  Unit Delay2/1 -> TimeUpdatePredict/1(uk)

== system v1_0_3_sim_fsfc/Optimization/Efficiency/Pin ==
  idq : Inport
  u : Inport  Port=2
  Add : Sum
  Demux : Demux  Outputs=2
  Demux1 : Demux  Outputs=2
  Gain : Gain  Gain=1.5
  Product : Product
  Product1 : Product
  Pin : Outport
  wires:
  Product/1 -> Add/1
  Product1/1 -> Add/2
  Add/1 -> Gain/1
  Gain/1 -> Pin/1
  Demux1/1 -> Product/1  "id"
  Demux1/2 -> Product1/1  "iq"
  Demux/1 -> Product/2  "vd"
  Demux/2 -> Product1/2  "vq"
  u/1 -> Demux/1
  idq/1 -> Demux1/1

== system v1_0_3_sim_fsfc/Optimization/Efficiency/Pout ==
  Omega_m : Inport
  idq : Inport  Port=2
  Pin : Inport  Port=3
  Add : Sum  Inputs=----+
  P_Cu : MATLAB Function  TreatAsAtomicUnit=on
  P_Fe : MATLAB Function  TreatAsAtomicUnit=on
  Pm : MATLAB Function  TreatAsAtomicUnit=on
  Ps : Gain  Gain=0.01
  Pout : Outport
  tag scope: T_Fe=global
  wires:
  idq/1 -> Pm/1(idq), P_Fe/1(idq), P_Cu/1(idq)
  Pin/1 -> Ps/1, Add/5
  Ps/1 -> Add/4
  Pm/1(Pm) -> Add/3
  P_Fe/1(P_Fe) -> Add/2
  P_Cu/1(P_Cu) -> Add/1
  Add/1 -> Pout/1
  Omega_m/1 -> Pm/2(Omega_m), P_Cu/2(Omega_m), P_Fe/2(Omega_m)
  P_Fe/2(T_Fe) -> [T_Fe]

== system v1_0_3_sim_fsfc/Optimization/Efficiency/Pout_hassan ==
  Xk_hat : Inport
  Pin : Inport  Port=2
  Add : Sum  Inputs=+--
  Add1 : Sum  Inputs=--+--
  P_Cu : MATLAB Function  TreatAsAtomicUnit=on
  P_Fe : MATLAB Function  TreatAsAtomicUnit=on
  Pe : MATLAB Function  TreatAsAtomicUnit=on
  Pm : MATLAB Function  TreatAsAtomicUnit=on
  Ps : Gain  Gain=0.01
  Pout_with_Pe : Outport
  Pout_with_CuFe : Outport  Port=2
  wires:
  Pin/1 -> Add1/3, Ps/1
  Pe/1(Pe) -> Add/1
  Pm/1(Pm) -> Add/2, Add1/2
  Ps/1 -> Add1/1, Add/3
  Add/1 -> Pout_with_Pe/1
  Xk_hat/1 -> Pe/1(Xk_hat), Pm/1(Xk_hat), P_Fe/1(Xk_hat), P_Cu/1(Xk_hat)
  P_Cu/1(P_Cu) -> Add1/4
  P_Fe/1(P_Fe) -> Add1/5
  Add1/1 -> Pout_with_CuFe/1

== matlab function v1_0_3_sim_fsfc/Optimization/Optim_maxi_eff ==
  data: Omega_m_opt output; Eff_opt output; Jc_min output; TL input; Rc parameter; Lambda_m parameter; L parameter; P parameter; Rs parameter; Tc parameter; Bv parameter; J parameter
function [Omega_m_opt, Eff_opt, Jc_min] = fcn(TL, Rc, Lambda_m, L, P, Rs, Tc, Bv, J)

Omega_m_min = 500; %rpm
Omega_m_max = 4000; %rmp

Omega_m_min = Omega_m_min*2*pi/60; %rad/s
Omega_m_max = Omega_m_max*2*pi/60; %rad/s

Omega_e_min = (P/2)*Omega_m_min*2*pi/60; %rad/s
Omega_e_max = (P/2)*Omega_m_max*2*pi/60; %rad/s

%% Method 1

% Eff_opt = 0;
% Omega_e_opt = Omega_m_max*P/2;
% for Omega_m = linspace(Omega_m_min, Omega_m_max, 1000)
%     Omega_e = Omega_m*P/2;
%      Eff_opt_calc = Calculate_Eff(Omega_e, idq, u, Rc, Lambda_m, L, P, Rs, Tc, Bv);
%      if Eff_opt_calc > Eff_opt
%          Eff_opt = Eff_opt_calc;
%          Omega_e_opt = Omega_e;
%      end
% end
%% Method 2
% Omega_m_a = Omega_m_min;
% Omega_e_a = Omega_m_a*P/2;
% 
% Omega_m_b = Omega_m_max;
% Omega_e_b = Omega_m_b*P/2;
% 
% a = Omega_e_a;
% b = Omega_e_b;
% tol = 1e-4;
% 
% for i = 1:500
%     c = (a+b)/2;
%     dEff_c = Calculate_dEff(c, idq, u, Rc, Lambda_m, L, P, Rs, Tc, Bv);
% 
%     if abs(b - a) < tol
%         break;
%     end
% 
%     if dEff_c > 0
%         a = c;
%     else
%         b = c;
%     end
% 
% end
% Compute optimal Omega_m_opt
% Omega_e_opt = (a + b) / 2;
%% Method 3
alpha = 1;
theta_e = 2*pi*100;
Eff_1min = 10;
Eff_1max = 100;

Omega_e = linspace(0, 0, 1000);
Eff = linspace(0, 0, 1000);
i = 0;
for Omega_m = linspace(Omega_m_min, Omega_m_max, 1000)
    i = i+1;
    Omega_e(i) = Omega_m*P/2;
    Eff(i) = Calculate_Eff(Omega_e(i), TL, Rc, Lambda_m, L, P, Rs, Tc, Bv, J);
end
[Eff_max, Eff_idx] = max(Eff);
Omega_e_opt = Omega_e(Eff_idx);
Omega_m_opt = Omega_e_opt * 2 / P;
Eff_opt = Eff_max;
Jc_min = 0;

if Eff_opt < 0.2
    Eff_opt = 0.2;
elseif Eff_opt > 1
    Eff_opt = 1;
end
Eff_opt = Eff_opt*100;



%% Calculate Pin
function Eff = Calculate_Eff(Omega_e, TL, Rc, Lambda_m, L, P, Rs, Tc, Bv, J)
    
    % dt = 0.00001;
    % Omega_e_dot = (Omega_e - Omega_e_dot)/dt;
    Omega_e_dot = 0;
    id = 0;

    Te = J*Omega_e_dot*2/P + TL + Bv*Omega_e*2/P;
    % iq = Te*4/(3*P*Lambda_m);

    iq = 4*Te*(Rc^2 + (L*Omega_e)^2)/(3*P*Lambda_m*Rc^2) + (Lambda_m*Omega_e - L*id*Omega_e)/Rc;

    % Calculate P_e
    P_e = Te*Omega_e*2/P;
    
    % Calculate P_Fe
    Iod_num = Rc^2*id + Rc*L*Omega_e*iq - L*Omega_e^2*Lambda_m;
    Iod_denum = Rc^2 + (L*Omega_e)^2;
    Iod = Iod_num/Iod_denum;
    
    Ioq_num = Rc*(Rc*iq - Lambda_m*Omega_e - L*id*Omega_e);
    Ioq_denum = Iod_denum;
    Ioq = Ioq_num/Ioq_denum;
    
    factor = (3/2)*(Omega_e^2/Rc);
    term1 = L*Ioq;
    term2 = Lambda_m + L*Iod;
    
    P_Fe = factor*(term1^2 + term2^2);
    
    % Calculate P_Cu
    factor_cu = (3/2)*Rs;
    term1_cu = Iod - (Omega_e*L*Ioq/Rc);
    term2_cu = Ioq + Omega_e*(Lambda_m + L*Iod)/Rc;
    
    P_Cu = factor_cu*(term1_cu^2 + term2_cu^2);
    
    % Calculate P_s
    P_s = 0.01*(P_Cu + P_Fe + P_e);
    
    % Calculate P_m
    term1_m = 4*Bv*Omega_e^2/P^2;
    term2_m = 2*Tc*Omega_e/P;
    
    P_m = term1_m + term2_m;
    
    % Calculate P_in
    P_in = P_Cu + P_Fe + P_e;
    % Calculate Efficiency
    Eff = (P_e - P_m - P_s)/P_in;
    % if Eff >= 1
    %     Eff = 1;
    % elseif Eff <= 0.1
    %     Eff = 10;
    % end
    % Eff = 100*Eff;


% %% Calculate dEfficiency
% function dEff_dWe = Calculate_dEff(Omega_e, TL, Rc, Lambda_m, L, P, Rs, Tc, Bv, J, Omega_e_dot)
% 
%     Eff1 = Calculate_Eff(Omega_e, TL, Rc, Lambda_m, L, P, Rs, Tc, Bv, J, Omega_e_dot);
%     Eff2 = Calculate_Eff(Omega_e, TL, Rc, Lambda_m, L, P, Rs, Tc, Bv, J, Omega_e_dot);
%     dOmega_e = Omega_e - Omega_e_dot;
%     dEff_dWe = (Eff2 - Eff1)/dOmega_e;


%% Calculate Omega_e_dot

== matlab function v1_0_3_sim_fsfc/SVPWM/v_alpha_beta2vabc(InvClarke) ==
  data: v_alph_beta input; vabc output
function vabc = fcn(v_alph_beta)

vabc = [
            1, 0;
            -1/2, sqrt(3)/2;
            -1/2, -sqrt(3)/2;
       ]*v_alph_beta;

== matlab function v1_0_3_sim_fsfc/Physical/iabc2idq/iabc2i_alpha_beta(FClarke) ==
  data: iabc input; i_alpha_beta output
function i_alpha_beta = fcn(iabc)

i_alpha_beta = 2/3*[
                        1, -0.5, -0.5;
                        0, sqrt(3)/2, -sqrt(3)/2;
                    ]*iabc;

== matlab function v1_0_3_sim_fsfc/Physical/iabc2idq/i_alpha_beta2idq(FPark) ==
  data: i_alpha_beta input; idq output; theta_e input
function idq = fcn(i_alpha_beta, theta_e)

idq = [
        cos(theta_e), sin(theta_e);
        -sin(theta_e), cos(theta_e);
      ]*i_alpha_beta;

== matlab function v1_0_3_sim_fsfc/Optimization/Optim._min_cost ==
  data: Omega_m_opt output; TL input; Eff_opt output; Rc parameter; Lambda_m parameter; L parameter; P parameter; Rs parameter; Tc parameter; Bv parameter; J parameter; Jc_min output
function [Omega_m_opt, Eff_opt, Jc_min] = fcn(TL, Rc, Lambda_m, L, P, Rs, Tc, Bv, J)

Omega_m_min = 500; %rpm
Omega_m_max = 4000; %rmp

Omega_m_min = Omega_m_min*2*pi/60; %rad/s
Omega_m_max = Omega_m_max*2*pi/60; %rad/s

Omega_e_min = (P/2)*Omega_m_min*2*pi/60; %rad/s
Omega_e_max = (P/2)*Omega_m_max*2*pi/60; %rad/s

%% Method 1
theta_e = 100*2*pi;
a_e = 0.16; % $/kWh (range 0.12$ to 0.16$)
a_t = 1.5625; % $/h -> Labor cost

Omega_e = linspace(0, 0, 1000);
Eff = linspace(0, 0, 1000);
Jc = linspace(0, 0, 1000);
i = 0;
for Omega_m = linspace(Omega_m_min, Omega_m_max, 1000)
    i = i+1;
    Omega_e(i) = Omega_m*P/2;
    [Eff(i), P_in] = Calculate_Eff(Omega_e(i), TL, Rc, Lambda_m, L, P, Rs, Tc, Bv, J);
    Ce = 27e-8*a_e;
    Ct = 27e-5*a_t;
    Jc(i) = P_in*theta_e/Omega_e(i)*Ce + theta_e/Omega_e(i)*Ct;
end
[Jc_min, Jc_idx] = min(Jc);
Omega_e_opt = Omega_e(Jc_idx);
Omega_m_opt = Omega_e_opt * 2 / P;
Eff_opt = Eff(Jc_idx);


if Eff_opt < 0.2
    Eff_opt = 0.2;
elseif Eff_opt > 1
    Eff_opt = 1;
end
Eff_opt = Eff_opt*100;




%% Calculate Pin
function [Eff, P_in] = Calculate_Eff(Omega_e, TL, Rc, Lambda_m, L, P, Rs, Tc, Bv, J)
    
    % dt = 0.00001;
    % Omega_e_dot = (Omega_e - Omega_e_dot)/dt;
    Omega_e_dot = 0;
    id = 0;

    Te = J*Omega_e_dot*2/P + TL + Bv*Omega_e*2/P;
    % iq = Te*4/(3*P*Lambda_m);

    iq = 4*Te*(Rc^2 + (L*Omega_e)^2)/(3*P*Lambda_m*Rc^2) + (Lambda_m*Omega_e - L*id*Omega_e)/Rc;

    % Calculate P_e
    P_e = Te*Omega_e*2/P;
    
    % Calculate P_Fe
    Iod_num = Rc^2*id + Rc*L*Omega_e*iq - L*Omega_e^2*Lambda_m;
    Iod_denum = Rc^2 + (L*Omega_e)^2;
    Iod = Iod_num/Iod_denum;
    
    Ioq_num = Rc*(Rc*iq - Lambda_m*Omega_e - L*id*Omega_e);
    Ioq_denum = Iod_denum;
    Ioq = Ioq_num/Ioq_denum;
    
    factor = (3/2)*(Omega_e^2/Rc);
    term1 = L*Ioq;
    term2 = Lambda_m + L*Iod;
    
    P_Fe = factor*(term1^2 + term2^2);
    
    % Calculate P_Cu
    factor_cu = (3/2)*Rs;
    term1_cu = Iod - (Omega_e*L*Ioq/Rc);
    term2_cu = Ioq + Omega_e*(Lambda_m + L*Iod)/Rc;
    
    P_Cu = factor_cu*(term1_cu^2 + term2_cu^2);
    
    % Calculate P_s
    P_s = 0.01*(P_Cu + P_Fe + P_e);
    
    % Calculate P_m
    term1_m = 4*Bv*Omega_e^2/P^2;
    term2_m = 2*Tc*Omega_e/P;
    
    P_m = term1_m + term2_m;
    
    % Calculate P_in
    P_in = P_Cu + P_Fe + P_e;
    % Calculate Efficiency
    Eff = (P_e - P_m - P_s)/(P_Cu + P_Fe + P_e);
    if Eff >= 1
        Eff = 1;
    elseif Eff <= 0.1
        Eff = 10;
    end
    Eff = 100*Eff;


% %% Calculate dEfficiency
% function dEff_dWe = Calculate_dEff(Omega_e, TL, Rc, Lambda_m, L, P, Rs, Tc, Bv, J, Omega_e_dot)
% 
%     Eff1 = Calculate_Eff(Omega_e, TL, Rc, Lambda_m, L, P, Rs, Tc, Bv, J, Omega_e_dot);
%     Eff2 = Calculate_Eff(Omega_e, TL, Rc, Lambda_m, L, P, Rs, Tc, Bv, J, Omega_e_dot);
%     dOmega_e = Omega_e - Omega_e_dot;
%     dEff_dWe = (Eff2 - Eff1)/dOmega_e;


%% Calculate Omega_e_dot

== matlab function v1_0_3_sim_fsfc/Estimation/EKF Estimation/EKF Estimation/MeasurementUpdateCorrect ==
  data: Zk input; Pk1_p input; Xk1_p input; Xk output; Pk output; Rd parameter
function [Xk, Pk] = fcn(Zk, Pk1_p, Xk1_p, Rd)

Hjk = [
        1, 0, 0, 0;
        0, 1, 0, 0;
        0, 0, 1, 0;
    ];


Kk = Pk1_p*Hjk'/(Hjk*Pk1_p*Hjk' + Rd);

Xk = Xk1_p + Kk*(Zk - Hjk*Xk1_p);

Pk = (eye(4) - Kk*Hjk)*Pk1_p;

== matlab function v1_0_3_sim_fsfc/Estimation/EKF Estimation/EKF Estimation/TimeUpdatePredict ==
  data: Pk1_p output; uk input; Xk1_p output; Xk input size=[4 1]; Pk input size=[4 4]; Qd parameter; Bv parameter; J parameter; Lambda_m parameter; P parameter; L parameter; R parameter; Ts parameter
function [Pk1_p, Xk1_p] = fcn(uk, Xk, Pk, Qd, Bv, J, Lambda_m, P, L, R, Ts)
id = Xk(1);
iq = Xk(2);
wm = Xk(3);

%Predict the state ahead
Ad = [
        -R/L, P/2*wm, 0, 0;
        -P/2*wm, -R/L, -P/2*Lambda_m/L, 0;
        0, 3*P/4*Lambda_m/J, -Bv/J, -1/J;
        0, 0, 0, 0;
    ];
Bd = [
        1/L, 0;
        0, 1/L;
        0, 0;
        0, 0;
    ];
Adk = eye(4) + Ts*Ad;
Bdk = Ts*Bd;

Xk1_p = Adk*Xk + Bdk*uk;

%Predict the error covariance ahead
Aj = [
        -R/L, P/2*wm, P/2*iq, 0;
        -P/2*wm, -R/L, -P/2*(Lambda_m/L+id), 0;
        0, 3*P/4*Lambda_m/J, -Bv/J, -1/J;
        0, 0, 0, 0;
    ];

Ajk = eye(4) + Ts*Aj;

Pk1_p = Ajk*Pk*Ajk' + Ts*Qd;

== matlab function v1_0_3_sim_fsfc/Controller/LoadCompensation ==
  data: TLe input; u output; P parameter; R parameter; Lambda_m parameter
function u = fcn(TLe, P, R, Lambda_m)

u = [
        0;
        4*R/(3*P*Lambda_m)*TLe;
    ];

== matlab function v1_0_3_sim_fsfc/Measurement/Measurement Noise/Measurement Noise  ==
  data: Nv output; Vid input; Viq input; Vwm input
function Nv = fcn(Vid, Viq, Vwm)

Amplitude = diag([Vid, Viq, Vwm]);

R = Amplitude^2;    % Variance of each component

Nv = sqrt(R)*randn(3,1); %For Inner Loop 3x1
% Nv2 = [
%         Nv3(1); 
%         Nv3(3);
%     ];       %For Integrator Loop 2x1, Id and Wm

== matlab function v1_0_3_sim_fsfc/Controller/NonLinearComp ==
  data: X input size=[3 1]; u output; P parameter; L parameter
function u = fcn(X, P, L)

id = X(1);
iq = X(2);
wm = X(3);

u = [
        -P/2*L*wm*iq;
        P/2*L*wm*id;
    ];

== matlab function v1_0_3_sim_fsfc/Optimization/Efficiency/Pout/P_Cu ==
  data: idq input; P_Cu output; Rc parameter; Lambda_m parameter; L parameter; P parameter; Rs parameter; Omega_m input
function P_Cu = fcn(idq, Rc, Lambda_m, L, P, Rs, Omega_m)

id = idq(1);
iq = idq(2);
Omega_e = Omega_m*P/2;

Iod_num = Rc^2*id + Rc*L*Omega_e*iq - L*Omega_e^2*Lambda_m;
Iod_denum = Rc^2 + (L*Omega_e)^2;
Iod = Iod_num/Iod_denum;

Ioq_num = Rc*(Rc*iq - Lambda_m*Omega_e - L*id*Omega_e);
Ioq_denum = Iod_denum;
Ioq = Ioq_num/Ioq_denum;

factor = (3/2)*Rs;
term1 = Iod - (Omega_e*L*Ioq/Rc);
term2 = Ioq + Omega_e*(Lambda_m + L*Iod)/Rc;

P_Cu = factor*(term1^2 + term2^2);

== matlab function v1_0_3_sim_fsfc/Optimization/Efficiency/Pout/P_Fe ==
  data: idq input; P_Fe output; Rc parameter; Lambda_m parameter; L parameter; P parameter; Omega_m input; T_Fe output
function [P_Fe, T_Fe] = fcn(idq, Rc, Lambda_m, L, P, Omega_m)

id = idq(1);
iq = idq(2);
Omega_e = Omega_m*P/2;

Iod_num = Rc^2*id + Rc*L*Omega_e*iq - L*Omega_e^2*Lambda_m;
Iod_denum = Rc^2 + (L*Omega_e)^2;
Iod = Iod_num/Iod_denum;

Ioq_num = Rc*(Rc*iq - Lambda_m*Omega_e - L*id*Omega_e);
Ioq_denum = Iod_denum;
Ioq = Ioq_num/Ioq_denum;

factor = (3/2)*(Omega_e^2/Rc);
term1 = L*Ioq;
term2 = Lambda_m + L*Iod;

P_Fe = factor*(term1^2 + term2^2);

factor1 = (3/2)*(Omega_e/Rc);
T_Fe = factor1*(term1^2 + term2^2)*P/2;

== matlab function v1_0_3_sim_fsfc/Optimization/Efficiency/Pout/Pm ==
  data: idq input; P parameter; Pm output; Tc parameter; Bv parameter; Omega_m input
function Pm = fcn(idq,P, Tc, Bv, Omega_m)

id = idq(1);
iq = idq(2);
Omega_e = Omega_m*P/2;


term1 = 4*Bv*Omega_e^2/P^2;
term2 = 2*Tc*Omega_e/P;

Pm = term1 + term2;

== matlab function v1_0_3_sim_fsfc/SVPWM/Calculate_T1T2T0 ==
  data: sector input; theta input; T1 output; V_ref input; T2 output; T0 output; Ts_pwm parameter; Vdc parameter
function [T1, T2, T0] = fcn(sector, theta, V_ref, Ts_pwm, Vdc)
    V_norm = sqrt(3)*V_ref/Vdc;
    theta_s = theta - (sector-1)*pi/3;

    T1 = V_norm*Ts_pwm*sin(pi/3-theta_s);
    T2 = V_norm*Ts_pwm*sin(theta_s);
    T0 = Ts_pwm - T1 - T2;

    if T0 < 0
        scale = Ts_pwm / (T1 + T2);
        T1 = T1 * scale;
        T2 = T2 * scale;
        T0 = 0;
    end

== matlab function v1_0_3_sim_fsfc/Optimization/Efficiency/Pout_hassan/P_Cu ==
  data: Xk_hat input; P_Cu output; Lambda_m parameter; L parameter; Rc parameter; P parameter; R parameter
function P_Cu = fcn(Xk_hat, Lambda_m, L, Rc, P, R)
id = Xk_hat(1);
iq = Xk_hat(2);
Omega_m = Xk_hat(3);
Omega_e = Omega_m*P/2;

factor = (3/2)*R;
denominator = (Rc^2 + (L*Omega_e)^2);

term1 = (Rc^2*id + Rc*L*Omega_e*iq - L*Omega_e^2*Lambda_m)/denominator;

term2 = Omega_e*L*(Rc*iq - Lambda_m*Omega_e - L*id*Omega_e)/denominator;

term3 = Rc*(Rc*iq - Lambda_m*Omega_e - L*id*Omega_e)/denominator;

term4 = (Omega_e/Rc)*(Lambda_m + L*term1);

P_Cu = factor * ((term1 - term2)^2 + (term3 + term4)^2);

== matlab function v1_0_3_sim_fsfc/PMSM DynModel/NonLinearTerm ==
  data: TL input; T_Fe input; X input; nonLinearTerm output; J parameter; P parameter
function nonLinearTerm = fcn(TL, T_Fe, X, J, P)

id = X(1);
iq = X(2);
wm = X(3);

nonLinearTerm = [
        0;
        0;
        -(TL + T_Fe)/J;
    ] + [
            P/2*wm*iq;
            -P/2*wm*id;
            0;
        ];

== matlab function v1_0_3_sim_fsfc/PMSM DynModel/PMSM Dynamic Model ==
  data: nonLinearTerm input; Noise input; u input; X input size=[3 1]; X output size=[3 1]; A parameter; B parameter; Ts parameter
function X = fcn(nonLinearTerm, Noise, u, X, A, B, Ts)
I3 = eye(3);
X = (I3 + Ts*A)*X + Ts*B*u + Ts*nonLinearTerm + Noise;

== matlab function v1_0_3_sim_fsfc/PMSM DynModel/Process Noise/Process Noise ==
  data: Nw output; Vid input; Viq input; Vwm input; Ts parameter
function Nw = fcn(Vid, Viq, Vwm, Ts)

Amplitude = diag([Vid, Viq, Vwm]);

Q = Amplitude^2;  % Variance of each component

Nw = sqrt(Ts*Q)*randn(3,1);

== matlab function v1_0_3_sim_fsfc/Optimization/Efficiency/Pout_hassan/P_Fe ==
  data: Xk_hat input; P_Fe output; Lambda_m parameter; L parameter; Rc parameter; P parameter
function P_Fe = fcn(Xk_hat, Lambda_m, L, Rc, P)
id = Xk_hat(1);
iq = Xk_hat(2);
Omega_m = Xk_hat(3);
Omega_e = Omega_m*P/2;

factor = (3/2)*Omega_e^2/Rc;

term1 = L*Rc*(Rc*iq - Lambda_m*Omega_e - L*id*Omega_e)/(Rc^2 + (L*Omega_e)^2);
term2 = Lambda_m + L*(Rc^2*id + Rc*L*Omega_e*iq - L*Omega_e^2*Lambda_m)/(Rc^2 + (L*Omega_e)^2);

P_Fe = factor * (term1^2 + term2^2);

== matlab function v1_0_3_sim_fsfc/Optimization/Efficiency/Pout_hassan/Pe ==
  data: Xk_hat input; Pe output; Lambda_m parameter; L parameter; Rc parameter; P parameter
function Pe = fcn(Xk_hat, Lambda_m, L, Rc, P)
id = Xk_hat(1);
iq = Xk_hat(2);
Omega_m = Xk_hat(3);
Omega_e = Omega_m*P/2;
factor = 3*P*Lambda_m*Rc*Omega_e/4;
numerator = Rc*iq - Lambda_m*Omega_e - L*id*Omega_e;
denomiator = Rc^2 + (L*Omega_e)^2;

Pe = factor*numerator/denomiator;

== matlab function v1_0_3_sim_fsfc/Optimization/Efficiency/Pout_hassan/Pm ==
  data: Xk_hat input; Pm output; Bv parameter; Tc parameter; P parameter
function Pm = fcn(Xk_hat, Bv, Tc, P)
% id = Xk_hat(1);
% iq = Xk_hat(2);
Omega_m = Xk_hat(3);
Omega_e = Omega_m*P/2;

Pm = (4/P^2)*Bv*Omega_e^2 + (2/P)*Tc*Omega_e;

== matlab function v1_0_3_sim_fsfc/Controller/Physical_Limiter ==
  data: u input; u_lim output; Vdc parameter
function u_lim = fcn(u, Vdc)
    vd = u(1);
    vq = u(2);
    V_max = Vdc/sqrt(3);

    V_mag = sqrt(vd^2 + vq^2);

    if V_mag > V_max
        scale = V_max / V_mag;
        vd_lim = vd * scale;
        vq_lim = vq * scale;
    else
        vd_lim = vd;
        vq_lim = vq;
    end
    u_lim  = [vd_lim; vq_lim];

== matlab function v1_0_3_sim_fsfc/Optimization/Efficiency/MATLAB Function ==
  data: Eff input; Eff output
function Eff = fcn(Eff)

if Eff < 0.2
    Eff = 0.2;
elseif Eff > 1
    Eff = 1;
end
Eff = Eff*100;

== matlab function v1_0_3_sim_fsfc/SVPWM/Calculate Sector ==
  data: v_alpha_beta input; sector output; theta output
function [sector, theta] = fcn(v_alpha_beta)
    theta = atan2(v_alpha_beta(2), v_alpha_beta(1));
    
    if theta < 0
        theta = theta + 2*pi;
    end

sector = floor(theta / (pi/3)) + 1;

== matlab function v1_0_3_sim_fsfc/SVPWM/Calculate_TaTbTc ==
  data: sector input; T1 input; T2 input; T0 input; Ta output; Tb output; Tc output; Ts_pwm parameter
function [Ta, Tb, Tc] = fcn(sector, T1, T2, T0, Ts_pwm)
    Ta = 0;
    Tb = 0;
    Tc = 0;
    switch sector
        case 1
            Ta = T1 + T2 + T0/2;
            Tb = T2 + T0/2;
            Tc = T0/2;
        case 2
            Ta = T1 + T0/2;
            Tb = T1 + T2 + T0/2;
            Tc = T0/2;
        case 3
            Ta = T0/2;
            Tb = T1 + T2 + T0/2;
            Tc = T2 + T0/2;
        case 4
            Ta = T0/2;
            Tb = T1 + T0/2;
            Tc = T1 + T2 + T0/2;
        case 5
            Ta = T2 + T0/2;
            Tb = T0/2;
            Tc = T1 + T2 + T0/2;
        case 6
            Ta = T1 + T2 + T0/2;
            Tb = T0/2;
            Tc = T1 + T0/2;
    end
    Ta = Ta/Ts_pwm;
    Tb = Tb/Ts_pwm;
    Tc = Tc/Ts_pwm;

== matlab function v1_0_3_sim_fsfc/SVPWM/Calculate Vref  ==
  data: V_alpha_beta input; V_ref output
function V_ref = fcn(V_alpha_beta)
    % V_ref = norm(V_alpha_beta);
    V_ref = sqrt(V_alpha_beta(1)^2 + V_alpha_beta(2)^2);

== matlab function v1_0_3_sim_fsfc/SVPWM/Generate PWM_ABC ==
  data: Ta input; Tb input; Tc input; carrier input; pwmA output; pwmB output; pwmC output; pwmAcom output; pwmBcom output; pwmCcom output
function [pwmA, pwmB, pwmC, pwmAcom, pwmBcom, pwmCcom] = fcn(Ta, Tb, Tc, carrier)

    pwmA = double(Ta >= carrier);
    pwmB = double(Tb >= carrier);
    pwmC = double(Tc >= carrier);
    
    pwmAcom = double(Ta < carrier);
    pwmBcom = double(Tb < carrier);
    pwmCcom = double(Tc < carrier);
    
    % if Tan > carrier
    %     pwmA = 1;
    %     pwmAcom = 0;
    % else
    %     pwmA =0;
    %     pwmAcom = 1;
    % end
    % 
    % if Tbn > carrier
    %     pwmB = 1;
    %     pwmBcom = 0;
    % else
    %     pwmB = 0;
    %     pwmBcom =1;
    % end
    % 
    % if Tcn > carrier
    %     pwmC = 1;
    %     pwmCcom = 0;
    % else
    %     pwmC =0;
    %     pwmCcom = 1;
    % end
